simulink model "cars"  (Simulink 9.3)
settings: Solver=VariableStepAuto  StartTime=0  StopTime=100  FixedStep=0.1  MinStep=0.01  RelTol=1e-3  AbsTol=1e-5  EnableMultiTasking=on
settings Model: Creator=yoriyuki  LastModifiedBy=khouloud.gaaloul
settings SolverCC: AutoInsertRateTranBlk=on
settings DataIOCC: ExternalInput=[Throttle, Brake]  FinalStateName=SavePoint  InitialState=SavePoint  SaveOperatingPoint=on  SignalLoggingSaveFormat=Dataset  SignalLogging=off  DSMLogging=off  StateSaveName=x
settings DebuggingCC: UnderspecifiedInitializationDetection=Simplified  MergeDetectMultiDrivingBlocksExec=error  FcnCallInpInsideContextMsg=error  AllowSymbolicDim=off
settings HardwareCC: ProdBitPerPointer=64  ProdBitPerSizeT=64  ProdBitPerPtrDiffT=64  ProdLargestAtomicFloat=Float  ProdIntDivRoundTo=Zero  ProdEndianess=LittleEndian  ProdWordSize=64  ProdHWDeviceType=Intel->x86-64 (Windows64)
settings ModelReferenceCC: PropagateSignalLabelsOutOfModel=on
settings GRTTargetCC: CombineOutputUpdateFcns=on  GRTInterface=off
settings ConfigComp: CovShowResultsExplorer=off

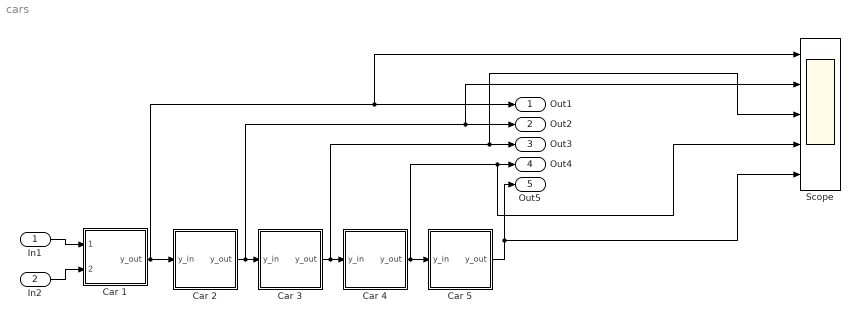
== system cars ==
  In1 : Inport
  In2 : Inport  Port=2
  Car 1 : Stateflow chart  TreatAsAtomicUnit=on
  Car 2 : Stateflow chart  TreatAsAtomicUnit=on
  Car 3 : Stateflow chart  TreatAsAtomicUnit=on
  Car 4 : Stateflow chart  TreatAsAtomicUnit=on
  Car 5 : Stateflow chart  TreatAsAtomicUnit=on
  Scope : Scope  NumInputPorts=5
  Out1 : Outport
  Out2 : Outport  Port=2
  Out3 : Outport  Port=3
  Out4 : Outport  Port=4
  Out5 : Outport  Port=5
  wires:
  Car 5/1(y_out) -> Scope/5, Out5/1
  Car 1/1(y_out) -> Scope/1, Out1/1, Car 2/1(y_in)
  Car 2/1(y_out) -> Scope/2, Out2/1, Car 3/1(y_in)
  Car 3/1(y_out) -> Scope/3, Out3/1, Car 4/1(y_in)
  Car 4/1(y_out) -> Car 5/1(y_in), Scope/4, Out4/1
  In1/1 -> Car 1/1(Throttle)
  In2/1 -> Car 1/2(Brake)

== stateflow chart Car 1 ==
  settings: updateMethod=CONTINUOUS
  state Run
    during:
    v_dot = -Throttle - Brake * v;
    y_dot = v;
    y_out = y;
  (default) -> Run
  data: Throttle input double; Brake input double; y local double =0; y_out output double; v local double =0
  data y settings: updateMethod=SF_CONTINUOUS_TIME_DATA
  data v settings: updateMethod=SF_CONTINUOUS_TIME_DATA

== stateflow chart Car 3 ==
  settings: updateMethod=CONTINUOUS
  state Chasing
    during:
    v_dot = 1;
    y_dot = -v;
    y_out = y;
  state Keeping
    during:
    y_dot = v;
    y_out = y;
  state Braking
    during:
    v_dot = -v;
    y_dot = -v;
    y_out = y;
  (default) -> Keeping
  Chasing -> Keeping : [y - y_in <= 10]
      | % [transition condition]{action}
  Keeping -> Chasing [order 1] : [y - y_in >=15]
  Braking -> Chasing : [y - y_in >= 20]
  Keeping -> Braking [order 2] : [y - y_in <=5]
  data: y_out output double; y local double =20; v local double =0; y_in input double
  data y settings: updateMethod=SF_CONTINUOUS_TIME_DATA
  data v settings: updateMethod=SF_CONTINUOUS_TIME_DATA
  data y_in settings: updateMethod=SF_CONTINUOUS_TIME_DATA

== stateflow chart Car 2 ==
  settings: updateMethod=CONTINUOUS
  state Chasing
    during:
    v_dot = 1;
    y_dot = -v;
    y_out = y;
  state Keeping
    during:
    y_dot = v;
    y_out = y;
  state Braking
    during:
    v_dot = -v;
    y_dot = -v;
    y_out = y;
  (default) -> Keeping
  Chasing -> Keeping : [y - y_in <= 10]
  Keeping -> Chasing [order 1] : [y - y_in >=15]
  Braking -> Chasing : [y - y_in >= 20]
  Keeping -> Braking [order 2] : [y - y_in <=5]
  data: y_out output double; y local double =10; v local double =0; y_in input double
  data y settings: updateMethod=SF_CONTINUOUS_TIME_DATA
  data v settings: updateMethod=SF_CONTINUOUS_TIME_DATA
  data y_in settings: updateMethod=SF_CONTINUOUS_TIME_DATA

== stateflow chart Car 4 ==
  settings: updateMethod=CONTINUOUS
  state Chasing
    during:
    v_dot = 1;
    y_dot = -v;
    y_out = y;
  state Keeping
    during:
    y_dot = v;
    y_out = y;
  state Braking
    during:
    v_dot = -v;
    y_dot = -v;
    y_out = y;
  (default) -> Keeping
  Chasing -> Keeping : [y - y_in <= 10]
      | % [transition condition]{action}
  Keeping -> Chasing [order 1] : [y - y_in >=15]
  Braking -> Chasing : [y - y_in >= 20]
  Keeping -> Braking [order 2] : [y - y_in <=5]
  data: y local double =30; v local double =0; y_in input double; y_out output double
  data y settings: updateMethod=SF_CONTINUOUS_TIME_DATA
  data v settings: updateMethod=SF_CONTINUOUS_TIME_DATA
  data y_in settings: updateMethod=SF_CONTINUOUS_TIME_DATA

== stateflow chart Car 5 ==
  settings: updateMethod=CONTINUOUS
  state Keeping
    during:
    y_dot = v;
    y_out = y;
  state Chasing
    during:
    v_dot = 1;
    y_dot = -v;
    y_out = y;
  state Braking
    during:
    v_dot = -v;
    y_dot = -v;
    y_out = y;
  (default) -> Keeping
  Chasing -> Keeping : [y - y_in <= 10]
      | % [transition condition]{action}
  Keeping -> Chasing [order 1] : [y - y_in >=15]
  Braking -> Chasing : [y - y_in >= 20]
  Keeping -> Braking [order 2] : [y - y_in <=5]
  data: y_out output double; y local double =40; v local double =0; y_in input double
  data y settings: updateMethod=SF_CONTINUOUS_TIME_DATA
  data v settings: updateMethod=SF_CONTINUOUS_TIME_DATA
  data y_in settings: updateMethod=SF_CONTINUOUS_TIME_DATA
